simulink model "tanque_cascata"  (Simulink 8.8)
settings: Solver=ode45  StartTime=0.0  StopTime=600  RelTol=1e-3  EnableMultiTasking=on
settings Model: Creator=Lideq2  LastModifiedBy=marcio
settings OptimizationCC: ExpressionDepthLimit=2147483647  InitFltsAndDblsToZero=on
settings DebuggingCC: SaveWithParameterizedLinksMsg=none  SolverPrmCheckMsg=warning  MultiTaskDSMMsg=warning  MultiTaskCondExecSysMsg=none
settings GRTTargetCC: TargetFcnLib=ansi_tfl_tmw.mat
settings ConfigComp: CovSFcnEnable=off

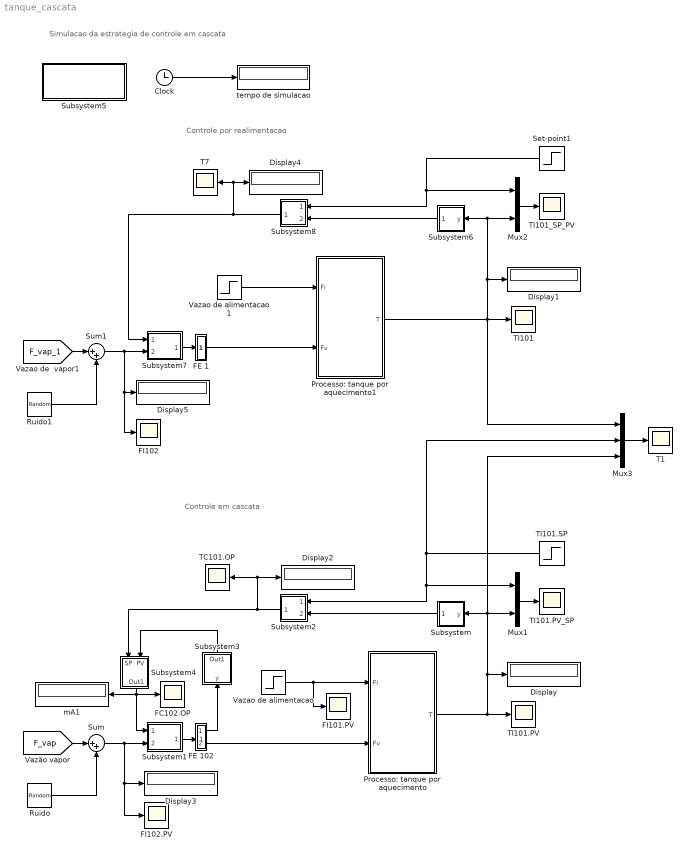
== system tanque_cascata ==
  note: Simulacao da estrategia de controle em cascata
  note: Controle em cascata
  note: Controle por realimentacao
  Clock : Clock
  Display{,1..5} (6 alike) : Display
  FC102.OP : Scope
  FE 1 : Subsystem
      mask Display: plot(-1*ones(1,21),[-2:0.2:2],zeros(1,11),[-1:0.2:1],1*ones(1,21),[-2:0.2:2])
  FE 102 : Subsystem
      mask Display: plot(-1*ones(1,21),[-2:0.2:2],zeros(1,11),[-1:0.2:1],1*ones(1,21),[-2:0.2:2])
  FI101.PV : Scope
  FI102 : Scope
  FI102.PV : Scope
  Mux1 : Mux  Inputs=2
  Mux2 : Mux  Inputs=2
  Mux3 : Mux  Inputs=3
  Processo: tanque por aquecimento : Subsystem  mask(Teste){Fi=1.5, Fv=0.4, T=57}
      mask prompts: Fi "Estado estacionário da vazão de alimentação do tanque [=] t/min"; Fv "Estado estacionário da vazão de vapor do tanque [=] t/min"; T "Temperatura de saída do tanque"
      mask help: Testando descrição
      mask init:
      | x = -1:.1:1;
      | y1 =  x;
      | y2 = -x;
      | 
      | x1 = zeros(1,3);
      | y3 = [0 1 7];
      | 
      | y4 = -1:.1:1;
      | r = sqrt(2);
      | x2 = sqrt(r^2-y4.^2);
      | x3 = -sqrt(r^2-y4.^2);
      | 
      | xs = -sqrt(2)-.5:0.1:sqrt(2)+.5;
      | ys = sin(10000*xs)/3-sqrt(2)-.3;
      | 
      | y1t = y1 + 3;
      | y2t = y2 + 3;
      | 
      | y4t = 2:.1:4;
      | x2t =  sqrt(r^2-(y4t-3).^2);
      | x3t = -sqrt(r^2-(y4t-3).^2);
      mask Help: TESTANDO HELP
      mask Display:
      | plot(x,y1,x,y2,x1,y3,x2,y4,x3,y4,xs,ys)
      | plot(x,y1t,x,y2t,x2t,y4t,x3t,y4t)
      | plot(sqrt(2)+0.5,0,-sqrt(2)-0.5,0)
  Processo: tanque por aquecimento1 : Subsystem  mask(Teste){Fi=1.5, Fv=0.4, T=57}
      mask prompts: Fi "Estado estacionário da vazão de alimentação do tanque [=] t/min"; Fv "Estado estacionário da vazão de vapor do tanque [=] t/min"; T "Temperatura de saída do tanque"
      mask help: Testando descrição
      mask init: same as tanque_cascata/Processo: tanque por aquecimento
      mask Help: TESTANDO HELP
      mask Display:
      | plot(x,y1,x,y2,x1,y3,x2,y4,x3,y4,xs,ys)
      | plot(x,y1t,x,y2t,x2t,y4t,x3t,y4t)
      | plot(sqrt(2)+0.5,0,-sqrt(2)-0.5,0)
  Ruido : RandomNumber  Variance=0.001  SampleTime=0
  Ruido1 : RandomNumber  Variance=0.001  SampleTime=0
  Set-point1 : Step  Time=50  Before=57  After=57*1.1  SampleTime=0
  Subsystem : Subsystem  mask(Transmissor){ymax=100, ymin=0}
      mask prompts: ymax "Valor máximo da variavel"; ymin "Valor minimo da variavel"
      mask init:
      | x = -1:.1:1;
      | r = 1;
      | y1 = sqrt(r^2 - x.^2);
      | y2 = -sqrt(r^2 - x.^2);
      mask Display:
      | disp('TT \n101')
      | plot(x,y1,x,y2)
  Subsystem1 : Subsystem  mask{Fmax=0.8, Fmin=0, talv=0.05}
      mask prompts: Fmax "Vazão máxima da valvula"; Fmin "Vazão minima da valvula"; talv "Dinâmica da valvula"
      mask init:
      | x= -1:.1:1;
      | 
      | y1=x;
      | y2=-x;
      | 
      | x1=[1,1];
      | y3=[1,-1];
      | x2=[-1,-1];
      | 
      | x3=[0,0,0];
      | y4=[0,1,2];
      | 
      | r=0.8;
      | x6= -r:.1:r;
      | y6 = sqrt(r^2-x6.^2)+2;
      | 
      | x5= [-r,r];
      | y5=[2,2];
      mask Display:
      | plot(x,y1,x,y2,x1,y3,x2,y3,x3,y4,x5,y5)
      | plot(x6,y6)
  Subsystem2 : Subsystem  mask(Controlador){AC=1, kc=2.4, tal_i=4.32, tal_d=0.05, BIAS=50, MODO=1}
      mask prompts: AC "Ação do controlador"; kc "Ganho do controlador"; tal_i "Constante de tempo integral"; tal_d "Constante de tempo derivativa"; BIAS "Posição da valvula em manual"; MODO "Modo de controle"
      mask init:
      | x = -1:.1:1;
      | r = 1;
      | y1 = sqrt(r^2 - x.^2);
      | y2 = -sqrt(r^2 - x.^2);
      mask Display:
      | disp('TC \n101')
      | plot(x,y1,x,y2)
  Subsystem3 : Subsystem  mask(Transmissor){ymax=0.4*2, ymin=0}
      mask prompts: ymax "Valor máximo da variavel"; ymin "Valor minimo da variavel"
      mask init:
      | x = -1:.1:1;
      | r = 1;
      | y1 = sqrt(r^2 - x.^2);
      | y2 = -sqrt(r^2 - x.^2);
      mask Display:
      | disp('FT\n102')
      | plot(x,y1,x,y2)
  Subsystem4 : Subsystem  mask(Controlador){AC=1, kc=3, tal_i=0.05, tal_d=0, BIAS=50, MODO=1}
      mask prompts: AC "Ação do controlador"; kc "Ganho do controlador"; tal_i "Constante de tempo integral"; tal_d "Constante de tempo derivativa"; BIAS "Posição da valvula em manual"; MODO "Modo de controle"
      mask init:
      | x = -1:.1:1;
      | r = 1;
      | y1 = sqrt(r^2 - x.^2);
      | y2 = -sqrt(r^2 - x.^2);
      mask Display:
      | disp('FC\n102')
      | plot(x,y1,x,y2)
  Subsystem5 : Subsystem
      settings: OpenFcn=save tanque
      mask Display: disp('Salvar \n dados')
  Subsystem6 : Subsystem  mask(Transmissor){ymax=100, ymin=0}
      mask prompts: ymax "Valor máximo da variavel"; ymin "Valor minimo da variavel"
      mask init:
      | x = -1:.1:1;
      | r = 1;
      | y1 = sqrt(r^2 - x.^2);
      | y2 = -sqrt(r^2 - x.^2);
      mask Display:
      | disp('TT\n101')
      | plot(x,y1,x,y2)
  Subsystem7 : Subsystem  mask{Fmax=0.8, Fmin=0, talv=0.05}
      mask prompts: Fmax "Vazão máxima da valvula"; Fmin "Vazão minima da valvula"; talv "Dinâmica da valvula"
      mask init:
      | x= -1:.1:1;
      | 
      | y1=x;
      | y2=-x;
      | 
      | x1=[1,1];
      | y3=[1,-1];
      | x2=[-1,-1];
      | 
      | x3=[0,0,0];
      | y4=[0,1,2];
      | 
      | r=0.8;
      | x6= -r:.1:r;
      | y6 = sqrt(r^2-x6.^2)+2;
      | 
      | x5= [-r,r];
      | y5=[2,2];
      mask Display:
      | plot(x,y1,x,y2,x1,y3,x2,y3,x3,y4,x5,y5)
      | plot(x6,y6)
  Subsystem8 : Subsystem  mask(Controlador){AC=1, kc=2.4, tal_i=4.32, tal_d=0.05, BIAS=50, MODO=1}
      mask prompts: AC "Ação do controlador"; kc "Ganho do controlador"; tal_i "Constante de tempo integral"; tal_d "Constante de tempo derivativa"; BIAS "Posição da valvula em manual"; MODO "Modo de controle"
      mask init:
      | x = -1:.1:1;
      | r = 1;
      | y1 = sqrt(r^2 - x.^2);
      | y2 = -sqrt(r^2 - x.^2);
      mask Display:
      | disp('TC\n101')
      | plot(x,y1,x,y2)
  Sum : Sum  Inputs=|++
  Sum1 : Sum  Inputs=|++
  T1 : Scope
  T7 : Scope
  TC101.OP : Scope
  TI101 : Scope
  TI101.PV : Scope
  TI101.PV_SP : Scope
  TI101.SP : Step  Time=50  Before=57  After=57*1.1  SampleTime=0
  TI101_SP_PV : Scope
  Vazao de alimentacao : Step  Time=300  Before=1.5  After=1.5*1.35  SampleTime=0
  Vazao de alimentacao1 : Step  Time=300  Before=1.5  After=1.5*1.35  SampleTime=0
  mA1 : Display
  tempo de simulacao : Display
  wires:
  Processo: tanque por aquecimento/1(T) -> TI101.PV/1, Display/1, Subsystem/1(y), Mux1/2, Mux3/3
  Vazao de alimentacao/1 -> Processo: tanque por aquecimento/1(Fi), FI101.PV/1
  Subsystem/1(Out1) -> Subsystem2/2(PV)
  Subsystem2/1(Out1) -> Display2/1, TC101.OP/1, Subsystem4/1(SP)
  Mux1/1 -> TI101.PV_SP/1
  TI101.SP/1 -> Subsystem2/1(SP), Mux1/1, Mux3/2
  Sum/1 -> Subsystem1/2(In2), Display3/1, FI102.PV/1
  [F_vap] -> Sum/1
  Ruido/1 -> Sum/2
  Subsystem3/1(Out1) -> Subsystem4/2(PV)
  Subsystem1/1(Out2) -> FE 102/1(In1)
  Subsystem4/1(Out1) -> FC102.OP/1, mA1/1, Subsystem1/1(In1)
  Clock/1 -> tempo de simulacao/1
  Processo: tanque por aquecimento1/1(T) -> Display1/1, Mux2/2, Subsystem6/1(y), TI101/1, Mux3/1
  Vazao de alimentacao1/1 -> Processo: tanque por aquecimento1/1(Fi)
  Subsystem6/1(Out1) -> Subsystem8/2(PV)
  Subsystem8/1(Out1) -> T7/1, Display4/1, Subsystem7/1(In1)
  Mux2/1 -> TI101_SP_PV/1
  Set-point1/1 -> Mux2/1, Subsystem8/1(SP)
  Sum1/1 -> FI102/1, Display5/1, Subsystem7/2(In2)
  [F_vap_1] -> Sum1/1
  Ruido1/1 -> Sum1/2
  Subsystem7/1(Out2) -> FE 1/1(In1)
  FE 1/1(Out2) -> Processo: tanque por aquecimento1/2(Fv)
  Mux3/1 -> T1/1
  FE 102/2(Out1) -> Processo: tanque por aquecimento/2(Fv)
  FE 102/1(Out2) -> Subsystem3/1(y)

== system tanque_cascata/FE 1 ==
  note: Placa de orifício
  In1 : Inport
  Out2 : Outport
  wires:
  In1/1 -> Out2/1

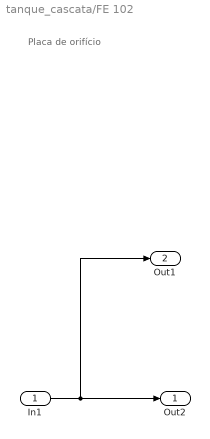
== system tanque_cascata/FE 102 ==
  note: Placa de orifício
  In1 : Inport
  Out2 : Outport
  Out1 : Outport  Port=2
  wires:
  In1/1 -> Out2/1, Out1/1

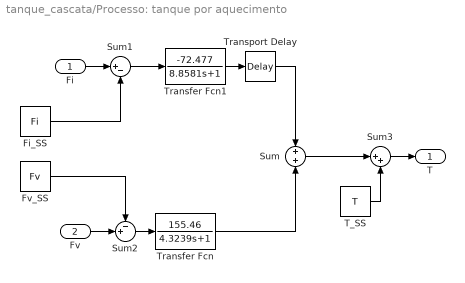
== system tanque_cascata/Processo: tanque por aquecimento ==
  Fi : Inport
  Fv : Inport  Port=2
  Fi_SS : Constant  Value=Fi
  Fv_SS : Constant  Value=Fv
  Sum : Sum  Inputs=+|+
  Sum1 : Sum  Inputs=|+-
  Sum2 : Sum  Inputs=-+|
  Sum3 : Sum  Inputs=|++
  T_SS : Constant  Value=T
  Transfer Fcn : TransferFcn  Numerator=[155.46]  Denominator=[4.3239 1]
  Transfer Fcn1 : TransferFcn  Numerator=[-72.477]  Denominator=[8.8581 1]
  Transport Delay : TransportDelay  DelayTime=2
  T : Outport
  wires:
  Sum/1 -> Sum3/1
  T_SS/1 -> Sum3/2
  Fi_SS/1 -> Sum1/2
  Fv_SS/1 -> Sum2/1
  Fi/1 -> Sum1/1
  Sum3/1 -> T/1
  Fv/1 -> Sum2/2
  Sum1/1 -> Transfer Fcn1/1
  Sum2/1 -> Transfer Fcn/1
  Transfer Fcn1/1 -> Transport Delay/1
  Transport Delay/1 -> Sum/1
  Transfer Fcn/1 -> Sum/2

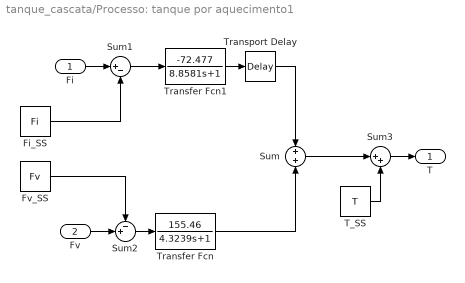
== system tanque_cascata/Processo: tanque por aquecimento1 ==
  Fi : Inport
  Fv : Inport  Port=2
  Fi_SS : Constant  Value=Fi
  Fv_SS : Constant  Value=Fv
  Sum : Sum  Inputs=+|+
  Sum1 : Sum  Inputs=|+-
  Sum2 : Sum  Inputs=-+|
  Sum3 : Sum  Inputs=|++
  T_SS : Constant  Value=T
  Transfer Fcn : TransferFcn  Numerator=[155.46]  Denominator=[4.3239 1]
  Transfer Fcn1 : TransferFcn  Numerator=[-72.477]  Denominator=[8.8581 1]
  Transport Delay : TransportDelay  DelayTime=2
  T : Outport
  wires:
  Transfer Fcn/1 -> Sum/2
  Transport Delay/1 -> Sum/1
  Transfer Fcn1/1 -> Transport Delay/1
  Sum2/1 -> Transfer Fcn/1
  Sum1/1 -> Transfer Fcn1/1
  Fv/1 -> Sum2/2
  Sum3/1 -> T/1
  Fi/1 -> Sum1/1
  Fv_SS/1 -> Sum2/1
  Fi_SS/1 -> Sum1/2
  T_SS/1 -> Sum3/2
  Sum/1 -> Sum3/1

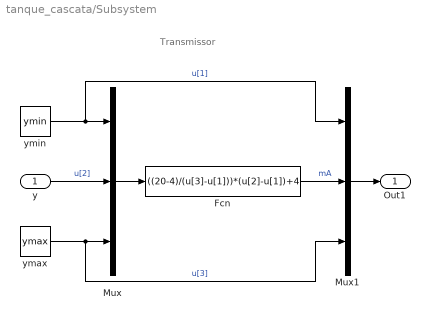
== system tanque_cascata/Subsystem ==
  note: Transmissor
  y : Inport
  Fcn : Fcn  Expr=((20-4)/(u[3]-u[1]))*(u[2]-u[1])+4
  Mux : Mux  Inputs=3
  Mux1 : Mux  Inputs=3
  ymax : Constant  Value=ymax
  ymin : Constant  Value=ymin
  Out1 : Outport
  wires:
  ymin/1 -> Mux/1, Mux1/1  "u[1]"
  y/1 -> Mux/2  "u[2]"
  ymax/1 -> Mux/3, Mux1/3  "u[3]"
  Mux/1 -> Fcn/1
  Fcn/1 -> Mux1/2  "mA"
  Mux1/1 -> Out1/1

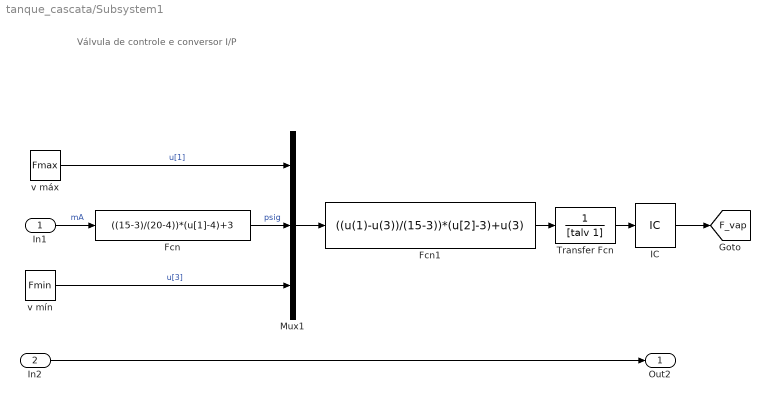
== system tanque_cascata/Subsystem1 ==
  note: Válvula de controle e conversor I/P
  In1 : Inport
  In2 : Inport  Port=2
  Fcn : Fcn  Expr=((15-3)/(20-4))*(u[1]-4)+3
  Fcn1 : Fcn  Expr=((u(1)-u(3))/(15-3))*(u[2]-3)+u(3)
  IC : InitialCondition  Value=0.4
  Mux1 : Mux  Inputs=3
  Transfer Fcn : TransferFcn  Denominator=[talv 1]
  v máx : Constant  Value=Fmax
  v mín : Constant  Value=Fmin
  Out2 : Outport
  tag scope: F_vap=global
  wires:
  Fcn/1 -> Mux1/2  "psig"
  In1/1 -> Fcn/1  "mA"
  Mux1/1 -> Fcn1/1
  v máx/1 -> Mux1/1  "u[1]"
  v mín/1 -> Mux1/3  "u[3]"
  In2/1 -> Out2/1
  Fcn1/1 -> Transfer Fcn/1
  IC/1 -> [F_vap]
  Transfer Fcn/1 -> IC/1

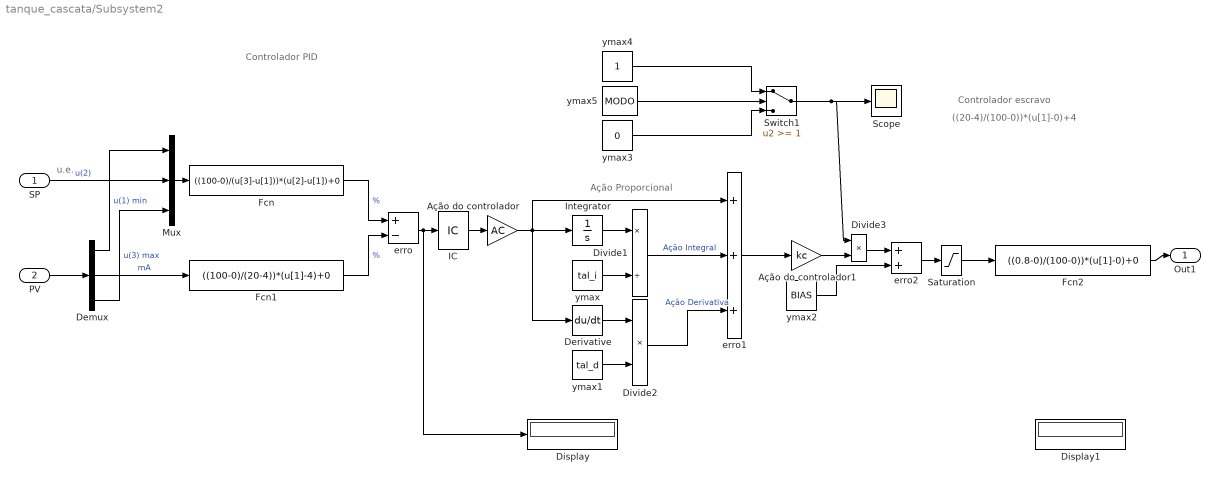
== system tanque_cascata/Subsystem2 ==
  note: Controlador PID
  note: u.e.
  note: Ação Proporcional
  note: ((20-4)/(100-0))*(u[1]-0)+4
  note: Controlador escravo
  SP : Inport
  PV : Inport  Port=2
  Ação do controlador : Gain  Gain=AC
  Ação do controlador1 : Gain  Gain=kc
  Demux : Demux  Outputs=3
  Derivative : Derivative
  Display : Display
  Display1 : Display
  Divide1 : Product  Inputs=*/
  Divide2 : Product
  Divide3 : Product
  Fcn : Fcn  Expr=((100-0)/(u[3]-u[1]))*(u[2]-u[1])+0
  Fcn1 : Fcn  Expr=((100-0)/(20-4))*(u[1]-4)+0
  Fcn2 : Fcn  Expr=((0.8-0)/(100-0))*(u[1]-0)+0
  IC : InitialCondition  Value=0
  Integrator : Integrator
  Mux : Mux  Inputs=3
  Saturation : Saturate  UpperLimit=100  LowerLimit=0
  Scope : Scope
  Switch1 : Switch  Threshold=1
  erro : Sum  Inputs=+-
  erro1 : Sum  Inputs=+++
  erro2 : Sum
  ymax : Constant  Value=tal_i
  ymax1 : Constant  Value=tal_d
  ymax2 : Constant  Value=BIAS
  ymax3 : Constant  Value=0
  ymax4 : Constant
  ymax5 : Constant  Value=MODO
  Out1 : Outport
  wires:
  PV/1 -> Demux/1
  SP/1 -> Mux/2  "u(2)"
  Demux/1 -> Mux/1  "u(1) min"
  Demux/3 -> Mux/3  "u(3) max"
  Mux/1 -> Fcn/1
  Demux/2 -> Fcn1/1  "mA"
  Fcn/1 -> erro/1  "%"
  Fcn1/1 -> erro/2  "%"
  erro/1 -> IC/1, Display/1
  Ação do controlador/1 -> Integrator/1, erro1/1, Derivative/1
  Integrator/1 -> Divide1/1
  ymax/1 -> Divide1/2
  Divide1/1 -> erro1/2  "Ação Integral"
  Derivative/1 -> Divide2/1
  ymax1/1 -> Divide2/2
  Divide2/1 -> erro1/3  "Ação Derivativa"
  erro1/1 -> Ação do controlador1/1
  ymax2/1 -> erro2/2
  erro2/1 -> Saturation/1
  ymax5/1 -> Switch1/2
  ymax4/1 -> Switch1/1
  ymax3/1 -> Switch1/3
  Divide3/1 -> erro2/1
  Ação do controlador1/1 -> Divide3/2
  Switch1/1 -> Divide3/1, Scope/1
  Fcn2/1 -> Out1/1
  IC/1 -> Ação do controlador/1
  Saturation/1 -> Fcn2/1

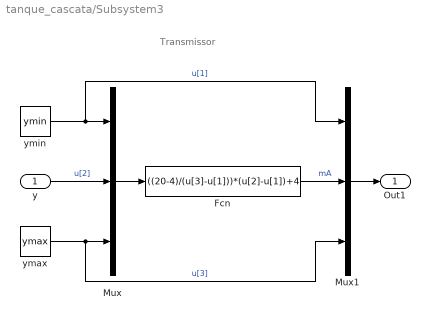
== system tanque_cascata/Subsystem3 ==
  note: Transmissor
  y : Inport
  Fcn : Fcn  Expr=((20-4)/(u[3]-u[1]))*(u[2]-u[1])+4
  Mux : Mux  Inputs=3
  Mux1 : Mux  Inputs=3
  ymax : Constant  Value=ymax
  ymin : Constant  Value=ymin
  Out1 : Outport
  wires:
  Mux1/1 -> Out1/1
  Fcn/1 -> Mux1/2  "mA"
  Mux/1 -> Fcn/1
  ymax/1 -> Mux1/3, Mux/3  "u[3]"
  y/1 -> Mux/2  "u[2]"
  ymin/1 -> Mux1/1, Mux/1  "u[1]"

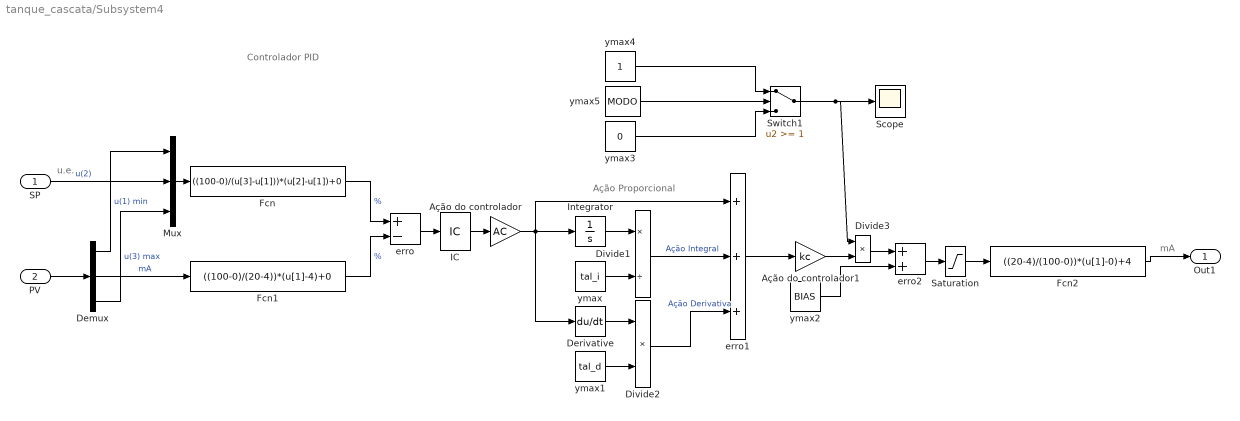
== system tanque_cascata/Subsystem4 ==
  note: mA
  note: Ação Proporcional
  note: u.e.
  note: Controlador PID
  SP : Inport
  PV : Inport  Port=2
  Ação do controlador : Gain  Gain=AC
  Ação do controlador1 : Gain  Gain=kc
  Demux : Demux  Outputs=3
  Derivative : Derivative
  Divide1 : Product  Inputs=*/
  Divide2 : Product
  Divide3 : Product
  Fcn : Fcn  Expr=((100-0)/(u[3]-u[1]))*(u[2]-u[1])+0
  Fcn1 : Fcn  Expr=((100-0)/(20-4))*(u[1]-4)+0
  Fcn2 : Fcn  Expr=((20-4)/(100-0))*(u[1]-0)+4
  IC : InitialCondition  Value=0
  Integrator : Integrator
  Mux : Mux  Inputs=3
  Saturation : Saturate  UpperLimit=100  LowerLimit=0
  Scope : Scope
  Switch1 : Switch  Threshold=1
  erro : Sum  Inputs=+-
  erro1 : Sum  Inputs=+++
  erro2 : Sum
  ymax : Constant  Value=tal_i
  ymax1 : Constant  Value=tal_d
  ymax2 : Constant  Value=BIAS
  ymax3 : Constant  Value=0
  ymax4 : Constant
  ymax5 : Constant  Value=MODO
  Out1 : Outport
  wires:
  IC/1 -> Ação do controlador/1
  Fcn2/1 -> Out1/1
  Saturation/1 -> Fcn2/1
  Switch1/1 -> Scope/1, Divide3/1
  Ação do controlador1/1 -> Divide3/2
  Divide3/1 -> erro2/1
  ymax3/1 -> Switch1/3
  ymax4/1 -> Switch1/1
  ymax5/1 -> Switch1/2
  erro2/1 -> Saturation/1
  ymax2/1 -> erro2/2
  erro1/1 -> Ação do controlador1/1
  Divide2/1 -> erro1/3  "Ação Derivativa"
  ymax1/1 -> Divide2/2
  Derivative/1 -> Divide2/1
  Divide1/1 -> erro1/2  "Ação Integral"
  ymax/1 -> Divide1/2
  Integrator/1 -> Divide1/1
  Ação do controlador/1 -> Derivative/1, erro1/1, Integrator/1
  erro/1 -> IC/1
  Fcn1/1 -> erro/2  "%"
  Fcn/1 -> erro/1  "%"
  Demux/2 -> Fcn1/1  "mA"
  Mux/1 -> Fcn/1
  Demux/3 -> Mux/3  "u(3) max"
  Demux/1 -> Mux/1  "u(1) min"
  SP/1 -> Mux/2  "u(2)"
  PV/1 -> Demux/1

== system tanque_cascata/Subsystem5 ==

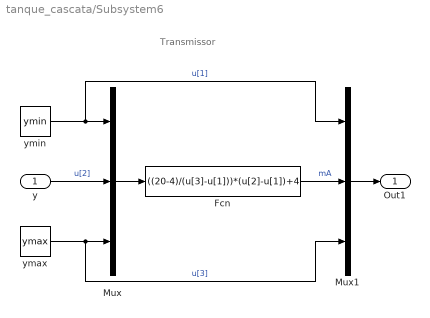
== system tanque_cascata/Subsystem6 ==
  note: Transmissor
  y : Inport
  Fcn : Fcn  Expr=((20-4)/(u[3]-u[1]))*(u[2]-u[1])+4
  Mux : Mux  Inputs=3
  Mux1 : Mux  Inputs=3
  ymax : Constant  Value=ymax
  ymin : Constant  Value=ymin
  Out1 : Outport
  wires:
  Mux1/1 -> Out1/1
  Fcn/1 -> Mux1/2  "mA"
  Mux/1 -> Fcn/1
  ymax/1 -> Mux1/3, Mux/3  "u[3]"
  y/1 -> Mux/2  "u[2]"
  ymin/1 -> Mux1/1, Mux/1  "u[1]"

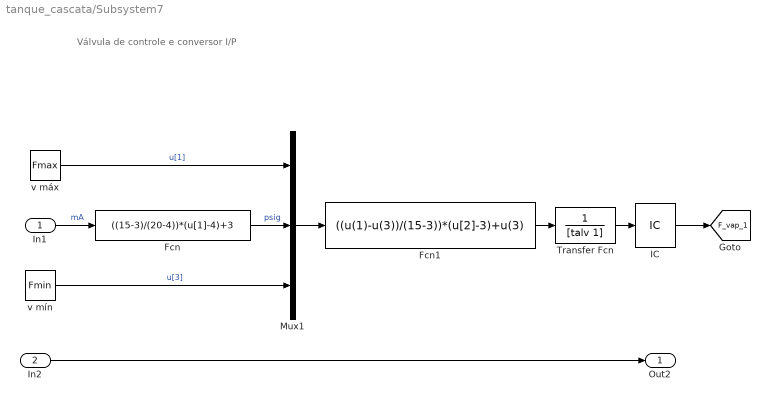
== system tanque_cascata/Subsystem7 ==
  note: Válvula de controle e conversor I/P
  In1 : Inport
  In2 : Inport  Port=2
  Fcn : Fcn  Expr=((15-3)/(20-4))*(u[1]-4)+3
  Fcn1 : Fcn  Expr=((u(1)-u(3))/(15-3))*(u[2]-3)+u(3)
  IC : InitialCondition  Value=0.4
  Mux1 : Mux  Inputs=3
  Transfer Fcn : TransferFcn  Denominator=[talv 1]
  v máx : Constant  Value=Fmax
  v mín : Constant  Value=Fmin
  Out2 : Outport
  tag scope: F_vap_1=global
  wires:
  Transfer Fcn/1 -> IC/1
  IC/1 -> [F_vap_1]
  Fcn1/1 -> Transfer Fcn/1
  In2/1 -> Out2/1
  v mín/1 -> Mux1/3  "u[3]"
  v máx/1 -> Mux1/1  "u[1]"
  Mux1/1 -> Fcn1/1
  In1/1 -> Fcn/1  "mA"
  Fcn/1 -> Mux1/2  "psig"

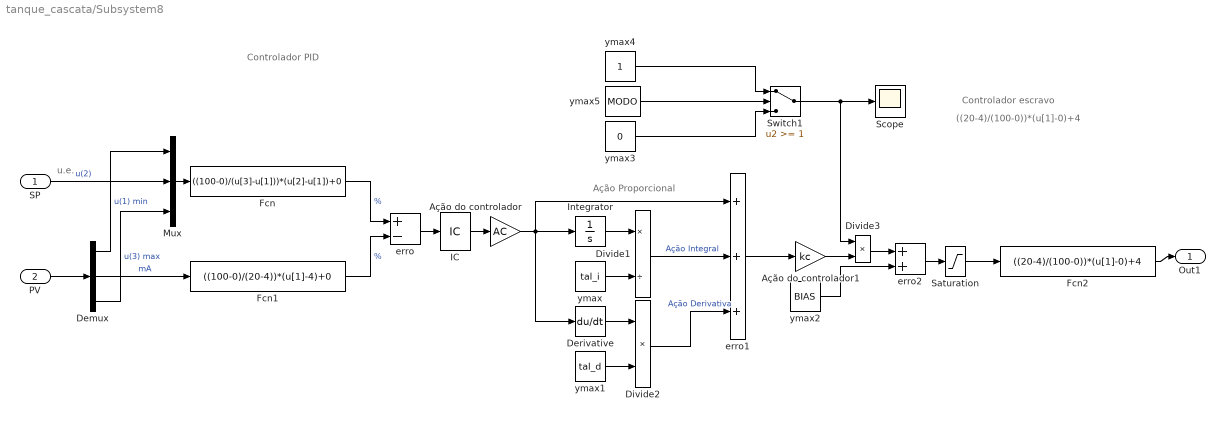
== system tanque_cascata/Subsystem8 ==
  note: Controlador escravo
  note: ((20-4)/(100-0))*(u[1]-0)+4
  note: Ação Proporcional
  note: u.e.
  note: Controlador PID
  SP : Inport
  PV : Inport  Port=2
  Ação do controlador : Gain  Gain=AC
  Ação do controlador1 : Gain  Gain=kc
  Demux : Demux  Outputs=3
  Derivative : Derivative
  Divide1 : Product  Inputs=*/
  Divide2 : Product
  Divide3 : Product
  Fcn : Fcn  Expr=((100-0)/(u[3]-u[1]))*(u[2]-u[1])+0
  Fcn1 : Fcn  Expr=((100-0)/(20-4))*(u[1]-4)+0
  Fcn2 : Fcn  Expr=((20-4)/(100-0))*(u[1]-0)+4
  IC : InitialCondition  Value=0
  Integrator : Integrator
  Mux : Mux  Inputs=3
  Saturation : Saturate  UpperLimit=100  LowerLimit=0
  Scope : Scope
  Switch1 : Switch  Threshold=1
  erro : Sum  Inputs=+-
  erro1 : Sum  Inputs=+++
  erro2 : Sum
  ymax : Constant  Value=tal_i
  ymax1 : Constant  Value=tal_d
  ymax2 : Constant  Value=BIAS
  ymax3 : Constant  Value=0
  ymax4 : Constant
  ymax5 : Constant  Value=MODO
  Out1 : Outport
  wires:
  Saturation/1 -> Fcn2/1
  IC/1 -> Ação do controlador/1
  Fcn2/1 -> Out1/1
  Switch1/1 -> Scope/1, Divide3/1
  Ação do controlador1/1 -> Divide3/2
  Divide3/1 -> erro2/1
  ymax3/1 -> Switch1/3
  ymax4/1 -> Switch1/1
  ymax5/1 -> Switch1/2
  erro2/1 -> Saturation/1
  ymax2/1 -> erro2/2
  erro1/1 -> Ação do controlador1/1
  Divide2/1 -> erro1/3  "Ação Derivativa"
  ymax1/1 -> Divide2/2
  Derivative/1 -> Divide2/1
  Divide1/1 -> erro1/2  "Ação Integral"
  ymax/1 -> Divide1/2
  Integrator/1 -> Divide1/1
  Ação do controlador/1 -> Derivative/1, erro1/1, Integrator/1
  erro/1 -> IC/1
  Fcn1/1 -> erro/2  "%"
  Fcn/1 -> erro/1  "%"
  Demux/2 -> Fcn1/1  "mA"
  Mux/1 -> Fcn/1
  Demux/3 -> Mux/3  "u(3) max"
  Demux/1 -> Mux/1  "u(1) min"
  SP/1 -> Mux/2  "u(2)"
  PV/1 -> Demux/1
